simulink model "SimulationComparison"  (R2022b)
settings: Solver=ode45  StartTime=0.0  StopTime=90000  FixedStep=1e-6  RelTol=1e-10  AbsTol=1e-10
settings Model: Creator=svens  LastModifiedBy=saraa
settings SolverCC: ZeroCrossAlgorithm=Adaptive
settings DebuggingCC: IgnoredZcDiagnostic=none

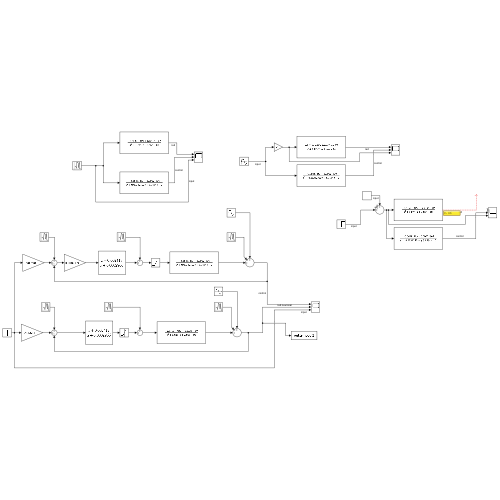
[thumbnail: Simulink's stored preview of the top-level diagram]
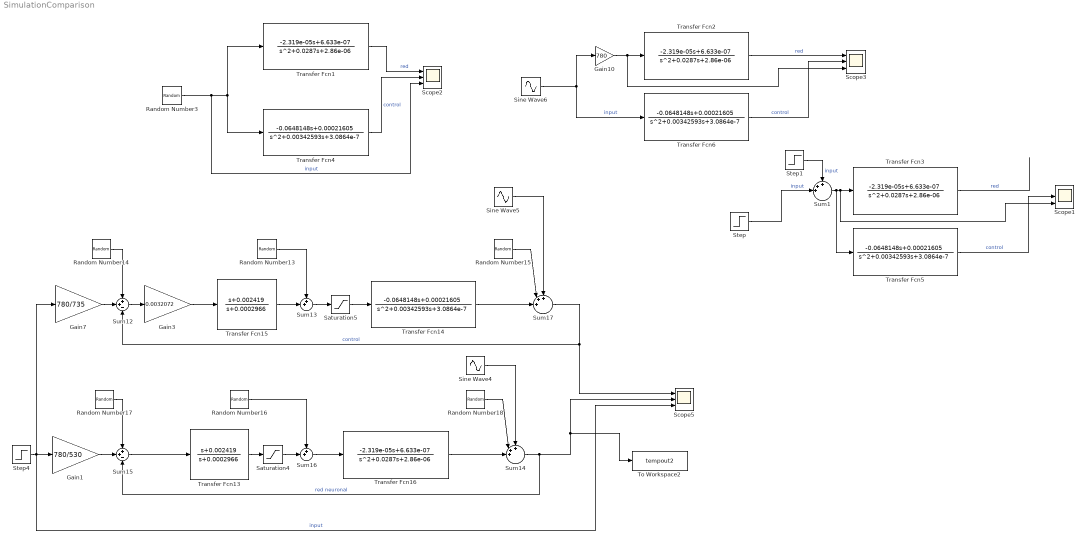
== system SimulationComparison ==
  Gain1 : Gain  Gain=780/530
  Gain10 : Gain  Gain=780
  Gain3 : Gain  Gain=0.0032072
  Gain7 : Gain  Gain=780/735
  Random Number{3,13..14,16..17} (5 alike) : RandomNumber  Variance=20  SampleTime=0.1
  Random Number15 : RandomNumber  Variance=20  SampleTime=7800
  Random Number18 : RandomNumber  Variance=20  SampleTime=7800
  Saturation4 : Saturate  UpperLimit=100000  LowerLimit=-10000
  Saturation5 : Saturate  UpperLimit=2  LowerLimit=0  LinearizeAsGain=off
  Scope{1..3,5} (4 alike) : Scope  NumInputPorts=3
  Sine Wave4 : Sin  Amplitude=6  Bias=25  Frequency=7.2e-5  SampleTime=0
  Sine Wave5 : Sin  Amplitude=6  Bias=25  Frequency=7.2e-5  SampleTime=0
  Sine Wave6 : Sin  SampleTime=0
  Step : Step  Time=500  SampleTime=0
  Step1 : Step  Time=50000  SampleTime=0
  Step4 : Step  After=780  SampleTime=0
  Sum1 : Sum  Inputs=+++||
  Sum12 : Sum  Inputs=++-
  Sum13 : Sum  Inputs=++|
  Sum14 : Sum  Inputs=+++||
  Sum15 : Sum  Inputs=++-
  Sum16 : Sum  Inputs=++|
  Sum17 : Sum  Inputs=+++||
  To Workspace2 : ToWorkspace  VariableName=tempout2  SaveFormat=Timeseries  SampleTime=-1
  Transfer Fcn{1..3,16} (4 alike) : TransferFcn  Numerator=[-2.319e-05 6.633e-07]  Denominator=[1 0.0287 2.86e-06]
  Transfer Fcn13 : TransferFcn  Numerator=[1 0.002419]  Denominator=[1 0.0002966]
  Transfer Fcn{4..6,14} (4 alike) : TransferFcn  Numerator=[-0.0648148 0.00021605]  Denominator=[1 0.00342593 3.0864e-7]
  Transfer Fcn15 : TransferFcn  Numerator=[1 0.002419]  Denominator=[1 0.0002966]
  wires:
  Sum13/1 -> Saturation5/1
  Random Number15/1 -> Sum17/2
  Gain3/1 -> Transfer Fcn15/1
  Sum17/1 -> Scope5/1, Sum12/3  "control"
  Random Number14/1 -> Sum12/1
  Transfer Fcn15/1 -> Sum13/2
  Gain7/1 -> Sum12/2
  Transfer Fcn14/1 -> Sum17/3
  Random Number17/1 -> Sum15/1
  Transfer Fcn16/1 -> Sum14/3
  Sum15/1 -> Transfer Fcn13/1
  Random Number16/1 -> Sum16/1
  Sine Wave5/1 -> Sum17/1
  Saturation4/1 -> Sum16/2
  Random Number18/1 -> Sum14/2
  Sum14/1 -> Scope5/2, To Workspace2/1, Sum15/3  "red neuronal"
  Random Number13/1 -> Sum13/1
  Sine Wave4/1 -> Sum14/1
  Sum16/1 -> Transfer Fcn16/1
  Step4/1 -> Gain1/1, Gain7/1, Scope5/3  "input"
  Saturation5/1 -> Transfer Fcn14/1
  Transfer Fcn13/1 -> Saturation4/1
  Sum12/1 -> Gain3/1
  Gain10/1 -> Transfer Fcn2/1, Scope3/3
  Random Number3/1 -> Scope2/3, Transfer Fcn1/1, Transfer Fcn4/1  "input"
  Transfer Fcn2/1 -> Scope3/1  "red"
  Transfer Fcn4/1 -> Scope2/2  "control"
  Transfer Fcn6/1 -> Scope3/2  "control"
  Sine Wave6/1 -> Gain10/1, Transfer Fcn6/1  "input"
  Transfer Fcn1/1 -> Scope2/1  "red"
  Gain1/1 -> Sum15/2
  Transfer Fcn3/1 -> ?  "red"
  Step/1 -> Sum1/3  "input"
  Transfer Fcn5/1 -> Scope1/2  "control"
  Step1/1 -> Sum1/1  "input"
  Sum1/1 -> Transfer Fcn5/1, Scope1/3, Transfer Fcn3/1
